simulink model "angle_estimator"  (Simulink 7.1)
settings: Solver=FixedStepDiscrete  StartTime=0.0  StopTime=10.0  FixedStep=0.001  RelTol=1e-3
undefined symbols (not defined in the file or in its folder): DiscIntNeverNeededParam, gaind, polesd, zerosd
libraries: dsPICdrivers x8, simulink x5
settings Model: Creator=Karthik  LastModifiedBy=Karthik
settings OptimizationCC: OptimizeModelRefInitCode=on  LifeSpan=1
settings HardwareCC: ProdBitPerInt=16  ProdEndianess=LittleEndian  ProdWordSize=16  ProdHWDeviceType=16-bit Generic
settings RTWCC: SystemTargetFile=dspic.tlc  TemplateMakefile=dspic_pic30_gcc.tmf  PostCodeGenCommand=dsPIC_Compile()  Description=Embedded Target for Microchip dsPIC (real-time)  ProcessScript=dspic_make_rtw_hook
settings CodeAppCC: IgnoreCustomStorageClasses=off
settings STFCustomTargetCC: ModelReferenceCompliant=off  IncludeMdlTerminateFcn=off  CombineOutputUpdateFcns=on  SuppressErrorStatus=on  ERTCustomFileBanners=on  SupportContinuousTime=off  SupportNonInlinedSFcns=off  SystemTargetFile=dspic.tlc
settings ERTTargetCC: ModelReferenceCompliant=off  CompOptLevelCompliant=off  IncludeMdlTerminateFcn=off  SuppressErrorStatus=on  ERTFirstTimeCompliant=off  ModelStepFunctionPrototypeControlCompliant=off  InlinedParameterPlacement=NonHierarchical  ERTSrcFileBannerTemplate=dsPIC_code_template.cgt  ERTHdrFileBannerTemplate=dsPIC_code_template.cgt  ERTDataSrcFileTemplate=dsPIC_code_template.cgt  ERTDataHdrFileTemplate=dsPIC_code_template.cgt  ERTCustomFileTemplate=dsPIC_main.tlc
settings CustomProperty: DataType=string  Value=F:\Matlab\bin\win32\gmake

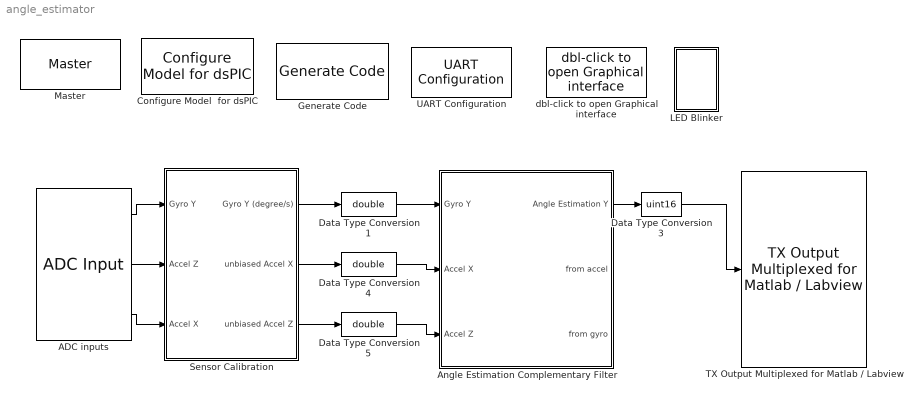
== system angle_estimator ==
  ADC inputs : dsPICdrivers/Peripheral I//O/ADC Input  Tag=dsPIC_ADC  Priority=5  ADC_TYPE=10 bits  ADC_MODE=Continuous sampling & get last channel value  NbrSampleStep=1  VoltRefpopup="AVdd  -  AVss"  OutFormatBitspopup=0000 00dd dddd dddd : Integer  InterruptPriority=6  ANCHANNELS=[0 1 2]  MaxName=ANmax = 1024  Rin=120  ADCS=0  SAMC=1  Temperature=25  DMAChannel=0  SampleTime=-1  Status="OK  |  Tsmp=1.667e-007 |  T/Channel=2.167e-006 |  Tall=6.500e-006"
  Angle Estimation Complementary Filter : Subsystem
  Configure Model  for dsPIC : dsPICdrivers/Simulink Configuration/Configure Model  for dsPIC
  Data Type Conversion1 : DataTypeConversion  OutDataTypeMode=double  OutDataType=sfix(16)  OutScaling=2^0  OutDataTypeStr=double
  Data Type Conversion3 : DataTypeConversion  OutDataTypeMode=uint16  OutDataType=sfix(16)  OutScaling=2^0  OutDataTypeStr=uint16
  Data Type Conversion4 : DataTypeConversion  OutDataTypeMode=double  OutDataType=sfix(16)  OutScaling=2^0  OutDataTypeStr=double
  Data Type Conversion5 : DataTypeConversion  OutDataTypeMode=double  OutDataType=sfix(16)  OutScaling=2^0  OutDataTypeStr=double
  Generate Code : dsPICdrivers/Simulink Configuration/Generate Code
  LED Blinker : Subsystem
  Master : dsPICdrivers/Master  Tag=dsPIC_MASTER  Priority=1  TimeStepType=Timer1  picType=30f4011  fcy=3e6  Quartz_33f=5e6  PLLActive_33f=off  fcyDesired_33f=0  tmr1="[1  2999  0]"  tmr1Info="Time Step : 0.001  ;   Error : 0%  PR1=2999"  tmr2345="[0  0  0  0]"  tmr2345cfg=[-1 -1 -1 -1]  IOautoConf=on  typePort="[ 0   0   0   0   0   0   0   0   0   0   0   0   0   0   0   0   8   8   8   0   0   0   0   0   0   0   0   0   0   0   0   0   0   0   0   0   0   0   0   0   0   0   0   0   0   5   4   0   0   0  10   0   0   0   0   0   0   0   0   0   0   0   0   0   0   0   0   0   0   0   0   0   0   0   0   0   0   0   0   0   0   0   0   0   0   0   0   0   0   0   0   0   0   0   0   0   0   0   0   0   0   0   0   0   0   0   0   0   0   0   0   0 ]"  TRIS="[ 65535  65535  65535  65531  65535  65535  65535 ]"  ADPCFG=0  MasterBusyPort=None  MasterOverloadPort=None  FOSC=HS  ClockSwitchMonitor=Both disabled  TempProtection_33f=TEMP_ON  FPBOR=PBOR_OFF  PWRT=PWRT_OFF  MCLR=MCLR_DIS  PowerSave=off  OverrideFcy=off  NewFcy=1e6
  Sensor Calibration : Subsystem
  TX Output Multiplexed for Matlab / Labview : dsPICdrivers/Serial PORT/TX Output Multiplexed for Matlab // Labview  Tag=dsPIC_TX_Multiplexed  Priority=5  UART=1  CleverSpreadingChk=on  CleverSpreading=1  CHANNEL=[0]  CHANNELBLOCKED=[]  CHANNELBLOCKED_BITEWISE=0  Status=OK
  UART Configuration : dsPICdrivers/Serial PORT/UART Configuration  Tag=dsPIC_config_UART  Priority=2  UART=1  proposed_BAUD=38400  ALT_TX_RX=on  InterruptTxWhen=When Transmit Buffer is empty  TXInterruptPri=1  TxBufferSize=32  TXEN=on  InterruptRxWhen=When Receive Buffer is full (contain 4 characters)  RXInterruptPri=2  RxBufferSize=32  BAUD=38400  UxBRG=4  Info="UxBRG = 4   ||  Real Baud : 37500   ||  % error : -2.3438  ||  max 3.75 Bytes / Step"  RealBaud=0
  dbl-click to open Graphical interface : dsPICdrivers/Serial PORT/dbl-click to open Graphical interface  SystemSampleTime=-1  Nothing=0
  wires:
  Data Type Conversion1/1 -> Angle Estimation Complementary Filter/1("Gyro Y ")
  Data Type Conversion4/1 -> Angle Estimation Complementary Filter/2(Accel X)
  Data Type Conversion5/1 -> Angle Estimation Complementary Filter/3(Accel Z)
  Sensor Calibration/1(Gyro Y (degree/s)) -> Data Type Conversion1/1
  Sensor Calibration/2(unbiased Accel X) -> Data Type Conversion4/1
  Sensor Calibration/3(unbiased Accel Z) -> Data Type Conversion5/1
  Angle Estimation Complementary Filter/1(Angle Estimation Y) -> Data Type Conversion3/1
  ADC inputs/1 -> Sensor Calibration/1(Gyro Y)
  ADC inputs/2 -> Sensor Calibration/2(Accel Z)
  ADC inputs/3 -> Sensor Calibration/3(Accel X)
  Data Type Conversion3/1 -> TX Output Multiplexed for Matlab / Labview/1

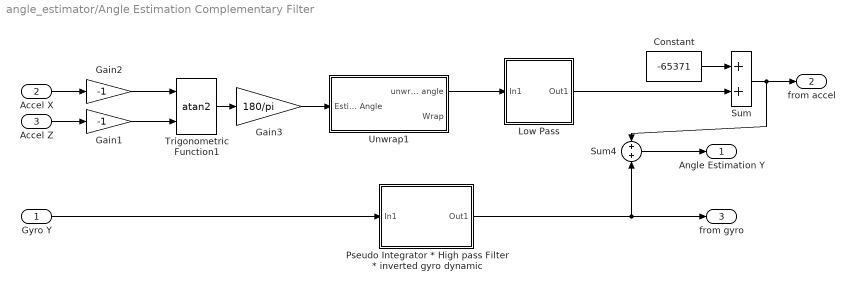
== system angle_estimator/Angle Estimation Complementary Filter ==
  "Gyro Y " : Inport
  Accel X : Inport  Port=2
  Accel Z : Inport  Port=3
  Constant : Constant  Value=-65371  OutDataType=sfix(16)  OutScaling=2^0
  Gain1 : Gain  Gain=-1  ParameterDataType=sfix(16)  ParameterScaling=2^0  OutDataType=sfix(16)  OutScaling=2^0
  Gain2 : Gain  Gain=-1  ParameterDataType=sfix(16)  ParameterScaling=2^0  OutDataType=sfix(16)  OutScaling=2^0
  Gain3 : Gain  Gain=180/pi  ParameterDataType=sfix(16)  ParameterScaling=2^0  OutDataTypeMode=Specify via dialog  OutDataType=float('double')  OutDataTypeStr=float('double')
  Low Pass : Subsystem  mask(DiscretizedZeroPole){Zeros=[], Poles=[-.5], Gain=.5, AbsTol=auto, SampleTime=.001, method=tustin, Wc=1}
      mask prompts: Zeros "Zeros (enter in s-main:)"; Poles "Poles (enter in s-domain:)"; Gain "Gain (enter in s-domain:)"; AbsTol "Absolute tolerance:"; SampleTime "Sample time:"; Wc "Critical Frequency (Hz):"
      mask help: Continuous mask uses c2d to transform parameters onto the Discrete Zero-Pole block inside.
      mask init:
      | st=SampleTime;
      | if length(st)>1
      |     st=SampleTime(1);
      | end
      | if(st>0)
      |     [zerosd,polesd,gaind] = sldiscutil('disczpk', {st,method,Wc,Zeros,Poles,Gain});
      | end	
      | s = get_param(gcb,'maskvalues');
      | zeross = s{1};
      | poless = s{2};
      | gainss = s{3};
      | %zerosc = eval(zeross);
      | %polesc = eval(poless);
      | %gainsc = eval(gainss);
      | sldiscutil('initzpkmask', st);
      | if(st==0)
      | set_param([gcb '/Zero Pole'], 'AbsoluteTolerance', AbsTol);
      | end
      mask StyleString: edit,edit,edit,edit,edit,popup(zoh|foh|tustin|prewarp|matched),edit
      mask CallbackString: |||||hidecrit|
      mask Display:
      | droots(zeross,poless,gainss)
      | text( 0.5, 1.0, method, 'verticalAlignment','top')
  Pseudo Integrator * High pass Filter * inverted gyro dynamic : Subsystem  mask(DiscretizedZeroPole){Zeros=[-314], Poles=[-.5], Gain=(1/314), AbsTol=auto, SampleTime=.001, method=tustin, Wc=1}
      mask prompts: Zeros "Zeros (enter in s-main:)"; Poles "Poles (enter in s-domain:)"; Gain "Gain (enter in s-domain:)"; AbsTol "Absolute tolerance:"; SampleTime "Sample time:"; Wc "Critical Frequency (Hz):"
      mask help: Continuous mask uses c2d to transform parameters onto the Discrete Zero-Pole block inside.
      mask init: same as angle_estimator/Angle Estimation Complementary Filter/Low Pass
      mask StyleString: edit,edit,edit,edit,edit,popup(zoh|foh|tustin|prewarp|matched),edit
      mask CallbackString: |||||hidecrit|
      mask Display:
      | droots(zeross,poless,gainss)
      | text( 0.5, 1.0, method, 'verticalAlignment','top')
  Sum : Sum  OutDataType=sfix(16)  OutScaling=2^0
  Sum4 : Sum  OutDataType=sfix(16)  OutScaling=2^0  SaturateOnIntegerOverflow=on
  Trigonometric Function1 : Trigonometry  Operator=atan2  OutputSignalType=real
  Unwrap1 : Subsystem
  Angle Estimation Y : Outport
  " from accel" : Outport  Port=2
  " from gyro" : Outport  Port=3
  wires:
  Pseudo Integrator * High pass Filter * inverted gyro dynamic/1(Out1) -> Sum4/2, " from gyro"/1
  Low Pass/1(Out1) -> Sum/2
  Accel X/1 -> Gain2/1
  Accel Z/1 -> Gain1/1
  Sum4/1 -> Angle Estimation Y/1
  "Gyro Y "/1 -> Pseudo Integrator * High pass Filter * inverted gyro dynamic/1(In1)
  Gain2/1 -> Trigonometric Function1/1
  Gain1/1 -> Trigonometric Function1/2
  Trigonometric Function1/1 -> Gain3/1
  Gain3/1 -> Unwrap1/1(Estimated Angle)
  Unwrap1/1(unwrap angle) -> Low Pass/1(In1)
  Constant/1 -> Sum/1
  Sum/1 -> " from accel"/1, Sum4/1

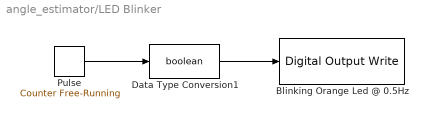
== system angle_estimator/LED Blinker ==
  Blinking Orange Led @ 0.5Hz : dsPICdrivers/Digital I//O/Digital Output Write  Tag=dsPIC_Digital_Output  Priority=5  PORT=D  Pin=[2]  Simultaneous=off  OrderingInOutPopup=None
  Data Type Conversion1 : DataTypeConversion  OutDataTypeMode=boolean  OutDataType=sfix(16)  OutScaling=2^0  OutDataTypeStr=boolean
  Pulse : simulink/Sources/Counter Free-Running  SystemSampleTime=-1  NumBits=1  tsamp=.25
  wires:
  Pulse/1 -> Data Type Conversion1/1
  Data Type Conversion1/1 -> Blinking Orange Led @ 0.5Hz/1

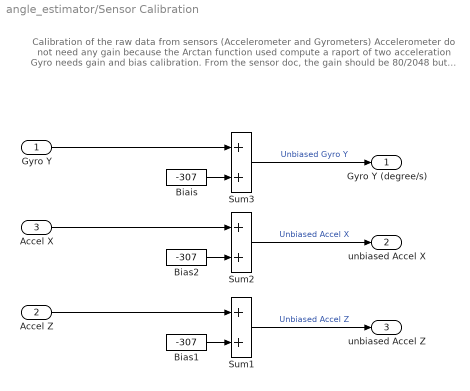
== system angle_estimator/Sensor Calibration ==
  note: Calibration of the raw data from sensors (Accelerometer and Gyrometers)
      | Accelerometer do not need any gain because the Arctan function used compute a raport of two acceleration
      | Gyro needs gain and bias calibration. From the sensor doc, the gain should be 80/2048 but...
  Gyro Y : Inport
  Accel Z : Inport  Port=2
  Accel X : Inport  Port=3
  "Biais " : Constant  Value=-307  OutDataType=sfix(16)  OutScaling=2^0
  Bias1 : Constant  Value=-307  OutDataType=sfix(16)  OutScaling=2^0
  Bias2 : Constant  Value=-307  OutDataType=sfix(16)  OutScaling=2^0
  Sum1 : Sum  OutDataType=sfix(16)  OutScaling=2^0
  Sum2 : Sum  OutDataType=sfix(16)  OutScaling=2^0
  Sum3 : Sum  OutDataType=sfix(16)  OutScaling=2^0
  Gyro Y (degree/s) : Outport
  unbiased Accel X : Outport  Port=2
  unbiased Accel Z : Outport  Port=3
  wires:
  "Biais "/1 -> Sum3/2
  Sum3/1 -> Gyro Y (degree/s)/1  "Unbiased Gyro Y"
  Sum2/1 -> unbiased Accel X/1  "Unbiased Accel X"
  Accel X/1 -> Sum2/1
  Sum1/1 -> unbiased Accel Z/1  "Unbiased Accel Z"
  Accel Z/1 -> Sum1/1
  Gyro Y/1 -> Sum3/1
  Bias2/1 -> Sum2/2
  Bias1/1 -> Sum1/2

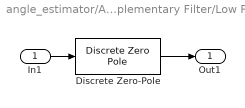
== system angle_estimator/Angle Estimation Complementary Filter/Low Pass ==
  In1 : Inport  OutDataType=sfix(16)  OutScaling=2^0
  Discrete Zero-Pole : DiscreteZeroPole  Zeros=zerosd  Poles=polesd  Gain=gaind  SampleTime=SampleTime
  Out1 : Outport  OutDataType=sfix(16)  OutScaling=2^0
  wires:
  In1/1 -> Discrete Zero-Pole/1
  Discrete Zero-Pole/1 -> Out1/1

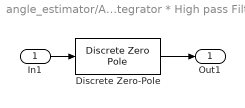
== system angle_estimator/Angle Estimation Complementary Filter/Pseudo Integrator * High pass Filter * inverted gyro dynamic ==
  In1 : Inport  OutDataType=sfix(16)  OutScaling=2^0
  Discrete Zero-Pole : DiscreteZeroPole  Zeros=zerosd  Poles=polesd  Gain=gaind  SampleTime=SampleTime
  Out1 : Outport  OutDataType=sfix(16)  OutScaling=2^0
  wires:
  In1/1 -> Discrete Zero-Pole/1
  Discrete Zero-Pole/1 -> Out1/1

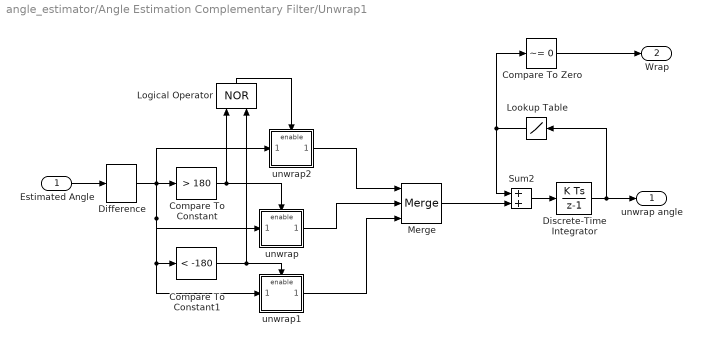
== system angle_estimator/Angle Estimation Complementary Filter/Unwrap1 ==
  Estimated Angle : Inport
  Compare To Constant : simulink/Logic and Bit Operations/Compare To Constant  SystemSampleTime=-1  relop=>  const=180  LogicOutDataTypeMode=uint8  ZeroCross=off
  Compare To Constant1 : simulink/Logic and Bit Operations/Compare To Constant  SystemSampleTime=-1  relop=<  const=-180  LogicOutDataTypeMode=uint8  ZeroCross=off
  Compare To Zero : simulink/Logic and Bit Operations/Compare To Zero  SystemSampleTime=-1  relop=~=  LogicOutDataTypeMode=uint8  ZeroCross=off
  Difference : simulink/Discrete/Difference  SystemSampleTime=-1  ICPrevInput=0.0  OutMin=[]  OutMax=[]  OutDataType=sfix(16)  OutScaling=2^-10  DoSatur=off
  Discrete-Time Integrator : DiscreteIntegrator  gainval=1000  SampleTime=-1  OutDataType=sfix(16)  OutScaling=2^0  ICPrevOutput=DiscIntNeverNeededParam  ICPrevScaledInput=DiscIntNeverNeededParam
  Logical Operator : Logic  Orientation=up  Operator=NOR  AllPortsSameDT=off  OutDataTypeMode=boolean  OutDataTypeStr=boolean
  Lookup Table : Lookup  Orientation=left  InputValues=[-500 -195 195]  Table=[+360 0 -360]  LookUpMeth=Use Input Below  OutDataType=sfix(16)  OutScaling=2^0
  Merge : Merge  Inputs=3
  Sum2 : Sum  OutDataType=sfix(16)  OutScaling=2^0
  unwrap : Subsystem  TreatAsAtomicUnit=on
  unwrap1 : Subsystem  TreatAsAtomicUnit=on
  unwrap2 : Subsystem  TreatAsAtomicUnit=on
  unwrap angle : Outport
  Wrap : Outport  Port=2
  wires:
  Compare To Zero/1 -> Wrap/1
  Lookup Table/1 -> Compare To Zero/1, Sum2/1
  Merge/1 -> Sum2/2
  Sum2/1 -> Discrete-Time Integrator/1
  Difference/1 -> Compare To Constant/1, unwrap/1(In1), Compare To Constant1/1, unwrap1/1(In1), unwrap2/1(In1)
  Compare To Constant/1 -> Logical Operator/1, unwrap/Enable
  Compare To Constant1/1 -> unwrap1/Enable, Logical Operator/2
  Logical Operator/1 -> unwrap2/Enable
  unwrap2/1(Out1) -> Merge/1
  unwrap/1(Out1) -> Merge/2
  unwrap1/1(Out1) -> Merge/3
  Estimated Angle/1 -> Difference/1
  Discrete-Time Integrator/1 -> Lookup Table/1, unwrap angle/1

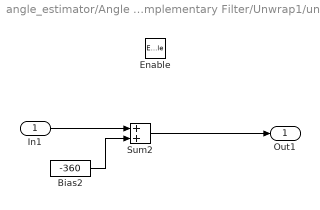
== system angle_estimator/Angle Estimation Complementary Filter/Unwrap1/unwrap ==
  In1 : Inport  OutDataType=sfix(16)  OutScaling=2^0
  Enable : EnablePort
  Bias2 : Constant  Value=-360  OutDataType=sfix(16)  OutScaling=2^0
  Sum2 : Sum  OutDataType=sfix(16)  OutScaling=2^0
  Out1 : Outport  OutDataType=sfix(16)  OutScaling=2^0
  wires:
  In1/1 -> Sum2/1
  Sum2/1 -> Out1/1
  Bias2/1 -> Sum2/2

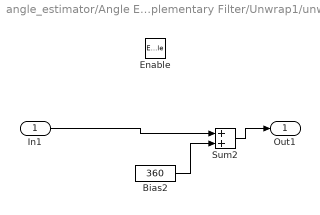
== system angle_estimator/Angle Estimation Complementary Filter/Unwrap1/unwrap1 ==
  In1 : Inport  OutDataType=sfix(16)  OutScaling=2^0
  Enable : EnablePort
  Bias2 : Constant  Value=360  OutDataType=sfix(16)  OutScaling=2^0
  Sum2 : Sum  OutDataType=sfix(16)  OutScaling=2^0
  Out1 : Outport  OutDataType=sfix(16)  OutScaling=2^0
  wires:
  In1/1 -> Sum2/1
  Bias2/1 -> Sum2/2
  Sum2/1 -> Out1/1

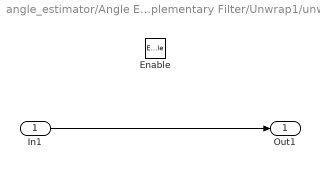
== system angle_estimator/Angle Estimation Complementary Filter/Unwrap1/unwrap2 ==
  In1 : Inport  OutDataType=sfix(16)  OutScaling=2^0
  Enable : EnablePort
  Out1 : Outport  OutDataType=sfix(16)  OutScaling=2^0
  wires:
  In1/1 -> Out1/1
